simulink model "planta_PROTEC_fornalha_LC"  (Simulink 8.8)
settings: Solver=ode3  StartTime=0.0  StopTime=800  FixedStep=tempo_amostragem  MaxStep=1e1  MinStep=1e-2  EnableMultiTasking=on
InitFcn:
  | planta_PROTEC_inicializacao
values from neighbouring files (symbols this model uses):
  Estado_Estacionario = [2 38.1987406965 21.9709981215 1.00092553605 3.07737941356 1.5 0.843438999559 0.0384242731301 0.118136727311 1.3 0.304251987406 0.577644341688 ... (188 elements, 1x188)]    [planta_PROTEC_estado_estacionario_inicial.mat]
  tempo_amostragem = 1e-2    (= 0.01)    [planta_PROTEC_inicializacao.m]
libraries: simulink_extras x6
(part 2 of 3)

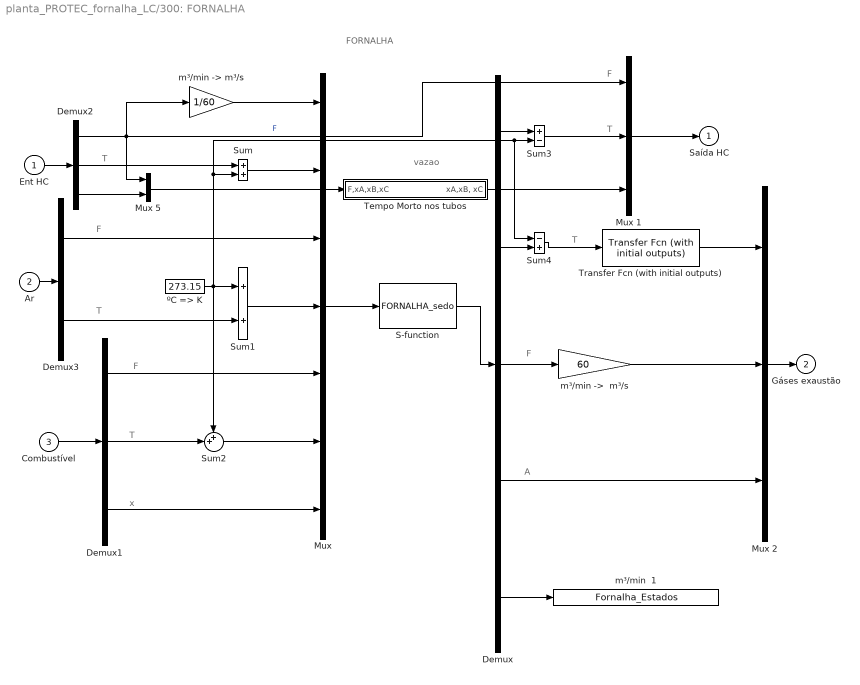
== system planta_PROTEC_fornalha_LC/300: FORNALHA ==
  note: T
  note: vazao
  note: FORNALHA
  note: T
  note: F
  note: T
  note: F
  note: A
  note: F
  note: T
  note: x
  note: F
  note: T
  Ent HC : Inport
  Ar : Inport  Port=2
  Combustível : Inport  Port=3
  "   m³/min  1" : ToWorkspace  VariableName=Fornalha_Estados  SampleTime=-1
      settings: Decimation=10
  Demux : Demux  Outputs=[ 1 1 1 1 26 ]
  Demux1 : Demux  Outputs=3
  Demux2 : Demux  Outputs=[ 1 1 3]
  Demux3 : Demux  Outputs=2
  Mux : Mux  Inputs=7
  Mux 1 : Mux  Inputs=3
  Mux 2 : Mux  Inputs=3
  Mux 5 : Mux  Inputs=[1 3]
  S-function : S-Function  FunctionName=FORNALHA_sedo  Parameters=Estado_Estacionario  SFunctionDeploymentMode=off  EnableBusSupport=off
  Sum : Sum  SaturateOnIntegerOverflow=on  InputSameDT=on  OutDataTypeStr=Inherit: Same as first input
  Sum1 : Sum  SaturateOnIntegerOverflow=on  InputSameDT=on  OutDataTypeStr=Inherit: Same as first input
  Sum2 : Sum  Inputs=++|  SaturateOnIntegerOverflow=on  InputSameDT=on  OutDataTypeStr=Inherit: Same as first input
  Sum3 : Sum  Inputs=+-  SaturateOnIntegerOverflow=on  InputSameDT=on  OutDataTypeStr=Inherit: Same as first input
  Sum4 : Sum  Inputs=-+  SaturateOnIntegerOverflow=on  InputSameDT=on  OutDataTypeStr=Inherit: Same as first input
  Tempo Morto nos tubos : Subsystem
  Transfer Fcn (with initial outputs) : simulink_extras/Additional Linear/Transfer Fcn (with initial outputs)  N=[1]  D="[1  1]"  Y0=Estado_Estacionario(40)  U0=Estado_Estacionario(40)
  "m³/min ->  m³/s" : Gain  Gain=60  SaturateOnIntegerOverflow=on  OutDataTypeStr=Inherit: Same as input  ParamDataTypeStr=Inherit: Same as input
  "m³/min -> m³/s" : Gain  Gain=1/60  SaturateOnIntegerOverflow=on  OutDataTypeStr=Inherit: Same as input  ParamDataTypeStr=Inherit: Same as input
  ºC => K : Constant  Value=273.15
  Saída HC : Outport
  Gáses exaustão : Outport  Port=2
  wires:
  S-function/1 -> Demux/1
  Mux/1 -> S-function/1
  ºC => K/1 -> Sum1/1, Sum2/1, Sum/2, Sum3/2, Sum4/1
  Sum2/1 -> Mux/6
  Sum1/1 -> Mux/4
  Sum/1 -> Mux/2
  Demux3/2 -> Sum1/2
  Demux1/2 -> Sum2/2
  Demux1/3 -> Mux/7
  Demux/1 -> Sum3/1
  Demux/2 -> Sum4/2
  Sum3/1 -> Mux 1/2
  Mux 1/1 -> Saída HC/1
  Sum4/1 -> Transfer Fcn (with initial outputs)/1
  Mux 2/1 -> Gáses exaustão/1
  Demux/4 -> Mux 2/3
  Demux/3 -> "m³/min ->  m³/s"/1
  Demux3/1 -> Mux/3
  Demux1/1 -> Mux/5
  Ent HC/1 -> Demux2/1
  Demux2/1 -> Mux 5/1, "m³/min -> m³/s"/1, Mux 1/1  "F"
  Tempo Morto nos tubos/1("xA,xB, xC") -> Mux 1/3
  Demux2/3 -> Mux 5/2
  Mux 5/1 -> Tempo Morto nos tubos/1(F,xA,xB,xC)
  Demux2/2 -> Sum/1
  Demux/5 -> "   m³/min  1"/1
  Transfer Fcn (with initial outputs)/1 -> Mux 2/1
  "m³/min -> m³/s"/1 -> Mux/1
  "m³/min ->  m³/s"/1 -> Mux 2/2
  Combustível/1 -> Demux1/1
  Ar/1 -> Demux3/1

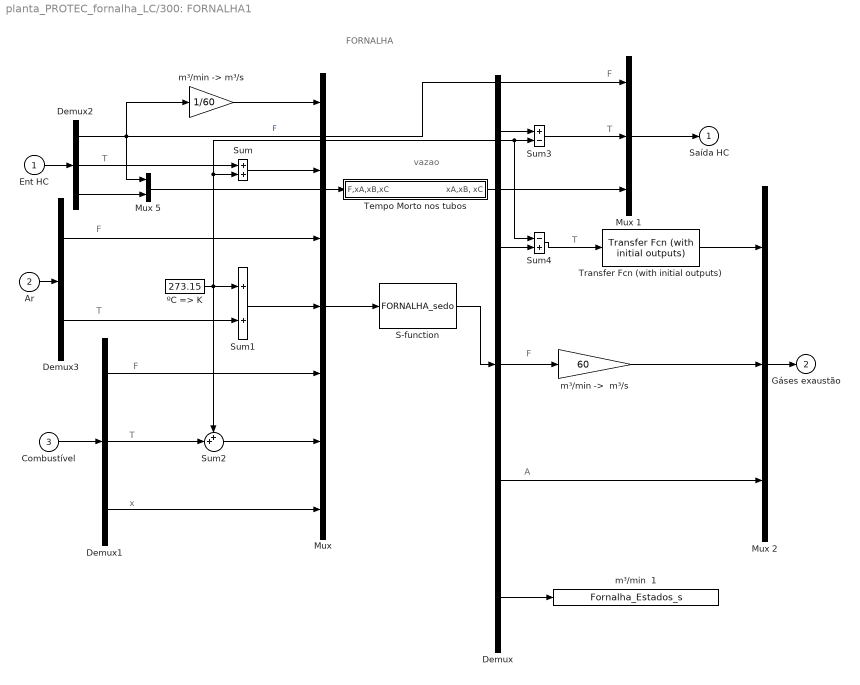
== system planta_PROTEC_fornalha_LC/300: FORNALHA1 ==
  note: T
  note: F
  note: x
  note: T
  note: F
  note: A
  note: F
  note: T
  note: F
  note: T
  note: FORNALHA
  note: vazao
  note: T
  Ent HC : Inport
  Ar : Inport  Port=2
  Combustível : Inport  Port=3
  "   m³/min  1" : ToWorkspace  VariableName=Fornalha_Estados_s  SampleTime=-1
      settings: Decimation=10
  Demux : Demux  Outputs=[ 1 1 1 1 26 ]
  Demux1 : Demux  Outputs=3
  Demux2 : Demux  Outputs=[ 1 1 3]
  Demux3 : Demux  Outputs=2
  Mux : Mux  Inputs=7
  Mux 1 : Mux  Inputs=3
  Mux 2 : Mux  Inputs=3
  Mux 5 : Mux  Inputs=[1 3]
  S-function : S-Function  FunctionName=FORNALHA_sedo  Parameters=Estado_Estacionario  SFunctionDeploymentMode=off  EnableBusSupport=off
  Sum : Sum  SaturateOnIntegerOverflow=on  InputSameDT=on  OutDataTypeStr=Inherit: Same as first input
  Sum1 : Sum  SaturateOnIntegerOverflow=on  InputSameDT=on  OutDataTypeStr=Inherit: Same as first input
  Sum2 : Sum  Inputs=++|  SaturateOnIntegerOverflow=on  InputSameDT=on  OutDataTypeStr=Inherit: Same as first input
  Sum3 : Sum  Inputs=+-  SaturateOnIntegerOverflow=on  InputSameDT=on  OutDataTypeStr=Inherit: Same as first input
  Sum4 : Sum  Inputs=-+  SaturateOnIntegerOverflow=on  InputSameDT=on  OutDataTypeStr=Inherit: Same as first input
  Tempo Morto nos tubos : Subsystem
  Transfer Fcn (with initial outputs) : simulink_extras/Additional Linear/Transfer Fcn (with initial outputs)  N=[1]  D="[1  1]"  Y0=Estado_Estacionario(40)  U0=Estado_Estacionario(40)
  "m³/min ->  m³/s" : Gain  Gain=60  SaturateOnIntegerOverflow=on  OutDataTypeStr=Inherit: Same as input  ParamDataTypeStr=Inherit: Same as input
  "m³/min -> m³/s" : Gain  Gain=1/60  SaturateOnIntegerOverflow=on  OutDataTypeStr=Inherit: Same as input  ParamDataTypeStr=Inherit: Same as input
  ºC => K : Constant  Value=273.15
  Saída HC : Outport
  Gáses exaustão : Outport  Port=2
  wires:
  Ar/1 -> Demux3/1
  Combustível/1 -> Demux1/1
  "m³/min ->  m³/s"/1 -> Mux 2/2
  "m³/min -> m³/s"/1 -> Mux/1
  Transfer Fcn (with initial outputs)/1 -> Mux 2/1
  Demux/5 -> "   m³/min  1"/1
  Demux2/2 -> Sum/1
  Mux 5/1 -> Tempo Morto nos tubos/1(F,xA,xB,xC)
  Demux2/3 -> Mux 5/2
  Tempo Morto nos tubos/1("xA,xB, xC") -> Mux 1/3
  Demux2/1 -> Mux 1/1, "m³/min -> m³/s"/1, Mux 5/1  "F"
  Ent HC/1 -> Demux2/1
  Demux1/1 -> Mux/5
  Demux3/1 -> Mux/3
  Demux/3 -> "m³/min ->  m³/s"/1
  Demux/4 -> Mux 2/3
  Mux 2/1 -> Gáses exaustão/1
  Sum4/1 -> Transfer Fcn (with initial outputs)/1
  Mux 1/1 -> Saída HC/1
  Sum3/1 -> Mux 1/2
  Demux/2 -> Sum4/2
  Demux/1 -> Sum3/1
  Demux1/3 -> Mux/7
  Demux1/2 -> Sum2/2
  Demux3/2 -> Sum1/2
  Sum/1 -> Mux/2
  Sum1/1 -> Mux/4
  Sum2/1 -> Mux/6
  ºC => K/1 -> Sum4/1, Sum3/2, Sum/2, Sum2/1, Sum1/1
  Mux/1 -> S-function/1
  S-function/1 -> Demux/1

== system planta_PROTEC_fornalha_LC/B 1 ==
  note: Bomba
  Sinal de entrada : Inport
  Sinal de saída : Outport
  wires:
  Sinal de entrada/1 -> Sinal de saída/1

== system planta_PROTEC_fornalha_LC/B 303 ==
  note: Bomba
  Sinal de entrada : Inport
  Sinal de saída : Outport
  wires:
  Sinal de entrada/1 -> Sinal de saída/1

== system planta_PROTEC_fornalha_LC/Clique duas vezes sobre  "?" para obter maiores informações  ==
  note: Autores:
      | Noaldo Leite Silva
      | Rômulo
  note: TROCADOR BITUBULAR EM CONTRA-CORRENTE.
      | Para rodar primeiro clique duas vezes no quadro que reinicializa os dados.
  note: Fonte:
  note: Simulação de uma fornalha
  note: Fonte: PROCESS CONTROL MODULES. Francis Doyle III
  note: Simulação de uma caldeira
  note: Fonte: Pellegrinetti, Gordon and Bentsman, Joseph. Nonlinear Control Oriented Boiler Modeling -
      | A Benchmark Problem for Controller Design. IEEE Transactions on Control System Technology,
      | Vol. 4, No. 1, January 1996
  note: Modelo do CSTR adaptado do Corripio, pg 471 a 474.
  note: Sugestões e críticas enviar para
      | e-mail: kalid@ufba.br
      |
      | Departamento de Engenharia Química da UFBA
      | Tel: (71) 3203.9811   ou   (71) 9188.3316
      |
      | Arquivos e outras informações em
      |
      | www.PEI.ufba.br
  note: Simulação de uma coluna de destilação
      | Fonte: S. Skogestad and M. Morari,
      | "Understanding the Dynamic Behavior of Distillation Columns'',
      | Ind. & Eng. Chem. Research, 27, 10, 1848-1862 (1988)
  note: Itens a desenvolver:
      | 1 Coluna de destilação: efeito da variação de pressão na separação
      | 2 Coluna de destilação: efeito da variação de pressão do vapor na entalpia do vapor para o refervedor
      | 3 Coluna de destilação: modelo fenomenológico com 3 componentes
      | 4 Ventilador de ar para fornalha
      | 5 Controle de pH no tanque de efluente
      | 6 Sistema de tratamento biológico no efluente
      | 7 No destilado instalar reator tubular
      | 8 Compressor de H2 e CO para reator tubular
      | 9 Melhor modelo de transferêcia de calor dos gases de exaustão na caldeira e no reator CSTR
      | 10 Modelo fenomenológico de bombas, ventiladores e exaustores
      | 11 Modelo fenomenológico de compressores

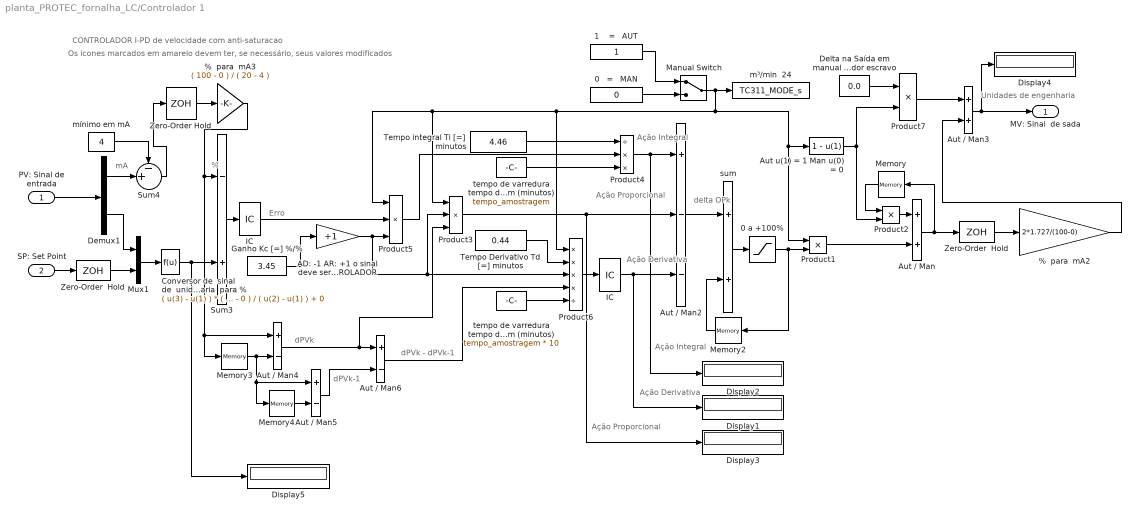
== system planta_PROTEC_fornalha_LC/Controlador 1 ==
  note: Ação
      | Proporcional
  note: Ação
      | Derivativa
  note: Ação
      | Integral
  note: Unidades
      | de
      | engenharia
  note: Ação
      | Integral
  note: Ação
      | Derivativa
  note: dPVk - dPVk-1
  note: dPVk
  note: dPVk-1
  note: delta
      | OPk
  note: Ação
      | Proporcional
  note: %
  note: mA
  note: CONTROLADOR I-PD de velocidade com anti-saturacao
  note: Os ícones marcados em amarelo devem ter, se necessário, seus valores modificados
  note: Erro
  PV: Sinal de entrada : Inport
  SP: Set Point : Inport  Port=2
  "   m³/min  24" : ToWorkspace  VariableName=TC311_MODE_s  SampleTime=-1
      settings: Decimation=10
  "  1    =   AUT" : Constant
  " IC" : InitialCondition  Value=0
  %  para  mA2 : Gain  Gain=2*1.727/(100-0)  SaturateOnIntegerOverflow=on  OutDataTypeStr=Inherit: Same as input  ParamDataTypeStr=Inherit: Same as input
  %  para  mA3 : Gain  Gain=( 100 - 0 ) / ( 20 - 4 )  SaturateOnIntegerOverflow=on  OutDataTypeStr=Inherit: Same as input  ParamDataTypeStr=Inherit: Same as input
  0   =   MAN : Constant  Value=0
  0 a +100% : Saturate  UpperLimit=100  LowerLimit=0  LinearizeAsGain=off
  "AD: -1 AR: +1 o sinal deve ser modificado para a  correta  AÇÃO  DO  CONTROLADOR   " : Gain  Gain=+1  SaturateOnIntegerOverflow=on  OutDataTypeStr=Inherit: Same as input  ParamDataTypeStr=Inherit: Same as input
  Aut / Man : Sum  SaturateOnIntegerOverflow=on  InputSameDT=on  OutDataTypeStr=Inherit: Same as first input
  Aut / Man2 : Sum  Inputs=+--  SaturateOnIntegerOverflow=on  InputSameDT=on  OutDataTypeStr=Inherit: Same as first input
  Aut / Man3 : Sum  SaturateOnIntegerOverflow=on  InputSameDT=on  OutDataTypeStr=Inherit: Same as first input
  Aut / Man4 : Sum  Inputs=+-  SaturateOnIntegerOverflow=on  InputSameDT=on  OutDataTypeStr=Inherit: Same as first input
  Aut / Man5 : Sum  Inputs=+-  SaturateOnIntegerOverflow=on  InputSameDT=on  OutDataTypeStr=Inherit: Same as first input
  Aut / Man6 : Sum  Inputs=+-  SaturateOnIntegerOverflow=on  InputSameDT=on  OutDataTypeStr=Inherit: Same as first input
  Aut u(1) = 1 Man u(0) = 0 : Fcn  Expr=1 - u(1)
  Conversor de  sinal de  unidades  de  engenharia  para % : Fcn  Expr=( u(3) - u(1) ) * ( 100 - 0 ) / ( u(2) - u(1) ) + 0
  Delta na Saída em manual do controlador [=] unidades de engenharia do SP do controlador escravo : Constant  Value=0.0
  Demux1 : Demux  Outputs=[ 1 2 ]
  Display{1..5} (5 alike) : Display
  Ganho Kc [=] %/% : Constant  Value=3.45
  IC : InitialCondition  Value=0
  Manual Switch : ManualSwitch
  Memory{,2..4} (4 alike) : Memory  X0=50  InheritSampleTime=on
  Mux1 : Mux  Inputs=[ 2 1 ]
  Product1 : Product  SaturateOnIntegerOverflow=on  RndMeth=Zero  InputSameDT=on  OutDataTypeStr=Inherit: Same as first input
  Product2 : Product  SaturateOnIntegerOverflow=on  RndMeth=Zero  InputSameDT=on  OutDataTypeStr=Inherit: Same as first input
  Product3 : Product  Inputs=3  SaturateOnIntegerOverflow=on  RndMeth=Zero  InputSameDT=on  OutDataTypeStr=Inherit: Same as first input
  Product4 : Product  Inputs=/**  SaturateOnIntegerOverflow=on  RndMeth=Zero  InputSameDT=on  OutDataTypeStr=Inherit: Same as first input
  Product5 : Product  Inputs=3  SaturateOnIntegerOverflow=on  RndMeth=Zero  InputSameDT=on  OutDataTypeStr=Inherit: Same as first input
  Product6 : Product  Inputs=****/  SaturateOnIntegerOverflow=on  RndMeth=Zero  InputSameDT=on  OutDataTypeStr=Inherit: Same as first input
  Product7 : Product  SaturateOnIntegerOverflow=on  RndMeth=Zero  InputSameDT=on  OutDataTypeStr=Inherit: Same as first input
  Sum3 : Sum  Inputs=-+  SaturateOnIntegerOverflow=on  InputSameDT=on  OutDataTypeStr=Inherit: Same as first input
  Sum4 : Sum  Inputs=-+|  SaturateOnIntegerOverflow=on  InputSameDT=on  OutDataTypeStr=Inherit: Same as first input
  Tempo Derivativo Td [=] minutos : Constant  Value=0.44
  Tempo integral Ti [=] minutos : Constant  Value=4.46
  Zero-Order  Hold : ZeroOrderHold  SampleTime=tempo_amostragem
  "Zero-Order  Hold " : ZeroOrderHold  SampleTime=tempo_amostragem
  "Zero-Order Hold " : ZeroOrderHold  SampleTime=tempo_amostragem
  mínimo em mA : Constant  Value=4
  sum : Sum  SaturateOnIntegerOverflow=on  InputSameDT=on  OutDataTypeStr=Inherit: Same as first input
  tempo de varredura tempo de amostragem (minutos) : Constant  Value=tempo_amostragem
  "tempo de varredura tempo de amostragem (minutos) " : Constant  Value=tempo_amostragem * 10
  MV: Sinal  de sada : Outport
  wires:
  Tempo Derivativo Td [=] minutos/1 -> Product6/2
  0   =   MAN/1 -> Manual Switch/2
  "  1    =   AUT"/1 -> Manual Switch/1
  Zero-Order  Hold/1 -> Mux1/2
  Demux1/2 -> Mux1/1
  Mux1/1 -> Conversor de  sinal de  unidades  de  engenharia  para %/1
  Aut / Man3/1 -> Display4/1, MV: Sinal  de sada/1
  %  para  mA2/1 -> Aut / Man3/2
  Product7/1 -> Aut / Man3/1
  Delta na Saída em manual do controlador [=] unidades de engenharia do SP do controlador escravo/1 -> Product7/1
  "Zero-Order  Hold "/1 -> %  para  mA2/1
  Sum4/1 -> "Zero-Order Hold "/1
  "Zero-Order Hold "/1 -> %  para  mA3/1
  Product3/1 -> Display3/1, Aut / Man2/2
  "AD: -1 AR: +1 o sinal deve ser modificado para a  correta  AÇÃO  DO  CONTROLADOR   "/1 -> Product5/3, Product3/2, Product6/3
  " IC"/1 -> Display1/1, Aut / Man2/3
  "tempo de varredura tempo de amostragem (minutos) "/1 -> Product6/5
  Aut / Man5/1 -> Aut / Man6/2
  Aut / Man4/1 -> Product3/3, Aut / Man6/1
  Conversor de  sinal de  unidades  de  engenharia  para %/1 -> Display5/1, Sum3/2
  Product6/1 -> " IC"/1
  Aut / Man6/1 -> Product6/4
  Memory4/1 -> Aut / Man5/2
  Memory3/1 -> Aut / Man4/2, Aut / Man5/1, Memory4/1
  Ganho Kc [=] %/%/1 -> "AD: -1 AR: +1 o sinal deve ser modificado para a  correta  AÇÃO  DO  CONTROLADOR   "/1
  IC/1 -> Product5/2
  0 a +100%/1 -> Product1/2, Memory2/1
  Memory2/1 -> sum/2
  sum/1 -> 0 a +100%/1
  Aut / Man2/1 -> sum/1
  Product4/1 -> Display2/1, Aut / Man2/1
  tempo de varredura tempo de amostragem (minutos)/1 -> Product4/3
  Tempo integral Ti [=] minutos/1 -> Product4/1
  Memory/1 -> Product2/1
  Aut / Man/1 -> "Zero-Order  Hold "/1, Memory/1
  Aut u(1) = 1 Man u(0) = 0/1 -> Product7/2, Product2/2
  Product2/1 -> Aut / Man/1
  Product1/1 -> Aut / Man/2
  Manual Switch/1 -> "   m³/min  24"/1, Product3/1, Product5/1, Product6/1, Aut u(1) = 1 Man u(0) = 0/1, Product1/1
  Product5/1 -> Product4/2
  Sum3/1 -> IC/1
  mínimo em mA/1 -> Sum4/1
  Demux1/1 -> Sum4/2
  %  para  mA3/1 -> Memory3/1, Aut / Man4/1, Sum3/1
  SP: Set Point/1 -> Zero-Order  Hold/1
  PV: Sinal de entrada/1 -> Demux1/1

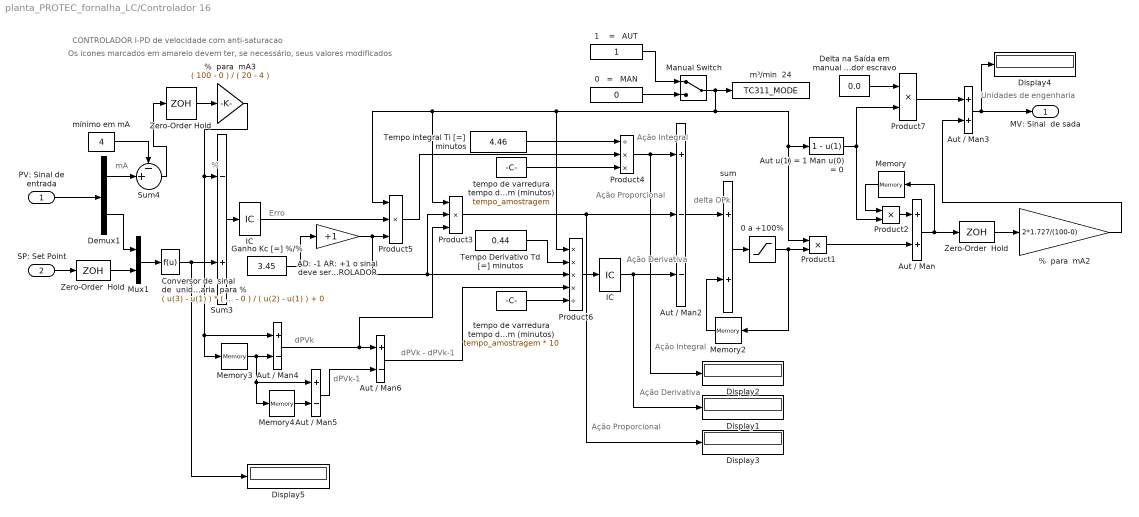
== system planta_PROTEC_fornalha_LC/Controlador 16 ==
  note: Erro
  note: Os ícones marcados em amarelo devem ter, se necessário, seus valores modificados
  note: CONTROLADOR I-PD de velocidade com anti-saturacao
  note: mA
  note: %
  note: Ação
      | Proporcional
  note: delta
      | OPk
  note: dPVk-1
  note: dPVk
  note: dPVk - dPVk-1
  note: Ação
      | Derivativa
  note: Ação
      | Integral
  note: Unidades
      | de
      | engenharia
  note: Ação
      | Integral
  note: Ação
      | Derivativa
  note: Ação
      | Proporcional
  PV: Sinal de entrada : Inport
  SP: Set Point : Inport  Port=2
  "   m³/min  24" : ToWorkspace  VariableName=TC311_MODE  SampleTime=-1
      settings: Decimation=10
  "  1    =   AUT" : Constant
  " IC" : InitialCondition  Value=0
  %  para  mA2 : Gain  Gain=2*1.727/(100-0)  SaturateOnIntegerOverflow=on  OutDataTypeStr=Inherit: Same as input  ParamDataTypeStr=Inherit: Same as input
  %  para  mA3 : Gain  Gain=( 100 - 0 ) / ( 20 - 4 )  SaturateOnIntegerOverflow=on  OutDataTypeStr=Inherit: Same as input  ParamDataTypeStr=Inherit: Same as input
  0   =   MAN : Constant  Value=0
  0 a +100% : Saturate  UpperLimit=100  LowerLimit=0  LinearizeAsGain=off
  "AD: -1 AR: +1 o sinal deve ser modificado para a  correta  AÇÃO  DO  CONTROLADOR   " : Gain  Gain=+1  SaturateOnIntegerOverflow=on  OutDataTypeStr=Inherit: Same as input  ParamDataTypeStr=Inherit: Same as input
  Aut / Man : Sum  SaturateOnIntegerOverflow=on  InputSameDT=on  OutDataTypeStr=Inherit: Same as first input
  Aut / Man2 : Sum  Inputs=+--  SaturateOnIntegerOverflow=on  InputSameDT=on  OutDataTypeStr=Inherit: Same as first input
  Aut / Man3 : Sum  SaturateOnIntegerOverflow=on  InputSameDT=on  OutDataTypeStr=Inherit: Same as first input
  Aut / Man4 : Sum  Inputs=+-  SaturateOnIntegerOverflow=on  InputSameDT=on  OutDataTypeStr=Inherit: Same as first input
  Aut / Man5 : Sum  Inputs=+-  SaturateOnIntegerOverflow=on  InputSameDT=on  OutDataTypeStr=Inherit: Same as first input
  Aut / Man6 : Sum  Inputs=+-  SaturateOnIntegerOverflow=on  InputSameDT=on  OutDataTypeStr=Inherit: Same as first input
  Aut u(1) = 1 Man u(0) = 0 : Fcn  Expr=1 - u(1)
  Conversor de  sinal de  unidades  de  engenharia  para % : Fcn  Expr=( u(3) - u(1) ) * ( 100 - 0 ) / ( u(2) - u(1) ) + 0
  Delta na Saída em manual do controlador [=] unidades de engenharia do SP do controlador escravo : Constant  Value=0.0
  Demux1 : Demux  Outputs=[ 1 2 ]
  Display{1..5} (5 alike) : Display
  Ganho Kc [=] %/% : Constant  Value=3.45
  IC : InitialCondition  Value=0
  Manual Switch : ManualSwitch
  Memory{,2..4} (4 alike) : Memory  X0=50  InheritSampleTime=on
  Mux1 : Mux  Inputs=[ 2 1 ]
  Product1 : Product  SaturateOnIntegerOverflow=on  RndMeth=Zero  InputSameDT=on  OutDataTypeStr=Inherit: Same as first input
  Product2 : Product  SaturateOnIntegerOverflow=on  RndMeth=Zero  InputSameDT=on  OutDataTypeStr=Inherit: Same as first input
  Product3 : Product  Inputs=3  SaturateOnIntegerOverflow=on  RndMeth=Zero  InputSameDT=on  OutDataTypeStr=Inherit: Same as first input
  Product4 : Product  Inputs=/**  SaturateOnIntegerOverflow=on  RndMeth=Zero  InputSameDT=on  OutDataTypeStr=Inherit: Same as first input
  Product5 : Product  Inputs=3  SaturateOnIntegerOverflow=on  RndMeth=Zero  InputSameDT=on  OutDataTypeStr=Inherit: Same as first input
  Product6 : Product  Inputs=****/  SaturateOnIntegerOverflow=on  RndMeth=Zero  InputSameDT=on  OutDataTypeStr=Inherit: Same as first input
  Product7 : Product  SaturateOnIntegerOverflow=on  RndMeth=Zero  InputSameDT=on  OutDataTypeStr=Inherit: Same as first input
  Sum3 : Sum  Inputs=-+  SaturateOnIntegerOverflow=on  InputSameDT=on  OutDataTypeStr=Inherit: Same as first input
  Sum4 : Sum  Inputs=-+|  SaturateOnIntegerOverflow=on  InputSameDT=on  OutDataTypeStr=Inherit: Same as first input
  Tempo Derivativo Td [=] minutos : Constant  Value=0.44
  Tempo integral Ti [=] minutos : Constant  Value=4.46
  Zero-Order  Hold : ZeroOrderHold  SampleTime=tempo_amostragem
  "Zero-Order  Hold " : ZeroOrderHold  SampleTime=tempo_amostragem
  "Zero-Order Hold " : ZeroOrderHold  SampleTime=tempo_amostragem
  mínimo em mA : Constant  Value=4
  sum : Sum  SaturateOnIntegerOverflow=on  InputSameDT=on  OutDataTypeStr=Inherit: Same as first input
  tempo de varredura tempo de amostragem (minutos) : Constant  Value=tempo_amostragem
  "tempo de varredura tempo de amostragem (minutos) " : Constant  Value=tempo_amostragem * 10
  MV: Sinal  de sada : Outport
  wires:
  PV: Sinal de entrada/1 -> Demux1/1
  SP: Set Point/1 -> Zero-Order  Hold/1
  %  para  mA3/1 -> Sum3/1, Aut / Man4/1, Memory3/1
  Demux1/1 -> Sum4/2
  mínimo em mA/1 -> Sum4/1
  Sum3/1 -> IC/1
  Product5/1 -> Product4/2
  Manual Switch/1 -> Product1/1, Aut u(1) = 1 Man u(0) = 0/1, Product6/1, Product5/1, Product3/1, "   m³/min  24"/1
  Product1/1 -> Aut / Man/2
  Product2/1 -> Aut / Man/1
  Aut u(1) = 1 Man u(0) = 0/1 -> Product2/2, Product7/2
  Aut / Man/1 -> Memory/1, "Zero-Order  Hold "/1
  Memory/1 -> Product2/1
  Tempo integral Ti [=] minutos/1 -> Product4/1
  tempo de varredura tempo de amostragem (minutos)/1 -> Product4/3
  Product4/1 -> Aut / Man2/1, Display2/1
  Aut / Man2/1 -> sum/1
  sum/1 -> 0 a +100%/1
  Memory2/1 -> sum/2
  0 a +100%/1 -> Memory2/1, Product1/2
  IC/1 -> Product5/2
  Ganho Kc [=] %/%/1 -> "AD: -1 AR: +1 o sinal deve ser modificado para a  correta  AÇÃO  DO  CONTROLADOR   "/1
  Memory3/1 -> Memory4/1, Aut / Man5/1, Aut / Man4/2
  Memory4/1 -> Aut / Man5/2
  Aut / Man6/1 -> Product6/4
  Product6/1 -> " IC"/1
  Conversor de  sinal de  unidades  de  engenharia  para %/1 -> Sum3/2, Display5/1
  Aut / Man4/1 -> Aut / Man6/1, Product3/3
  Aut / Man5/1 -> Aut / Man6/2
  "tempo de varredura tempo de amostragem (minutos) "/1 -> Product6/5
  " IC"/1 -> Aut / Man2/3, Display1/1
  "AD: -1 AR: +1 o sinal deve ser modificado para a  correta  AÇÃO  DO  CONTROLADOR   "/1 -> Product6/3, Product3/2, Product5/3
  Product3/1 -> Aut / Man2/2, Display3/1
  "Zero-Order Hold "/1 -> %  para  mA3/1
  Sum4/1 -> "Zero-Order Hold "/1
  "Zero-Order  Hold "/1 -> %  para  mA2/1
  Delta na Saída em manual do controlador [=] unidades de engenharia do SP do controlador escravo/1 -> Product7/1
  Product7/1 -> Aut / Man3/1
  %  para  mA2/1 -> Aut / Man3/2
  Aut / Man3/1 -> MV: Sinal  de sada/1, Display4/1
  Mux1/1 -> Conversor de  sinal de  unidades  de  engenharia  para %/1
  Demux1/2 -> Mux1/1
  Zero-Order  Hold/1 -> Mux1/2
  "  1    =   AUT"/1 -> Manual Switch/1
  0   =   MAN/1 -> Manual Switch/2
  Tempo Derivativo Td [=] minutos/1 -> Product6/2

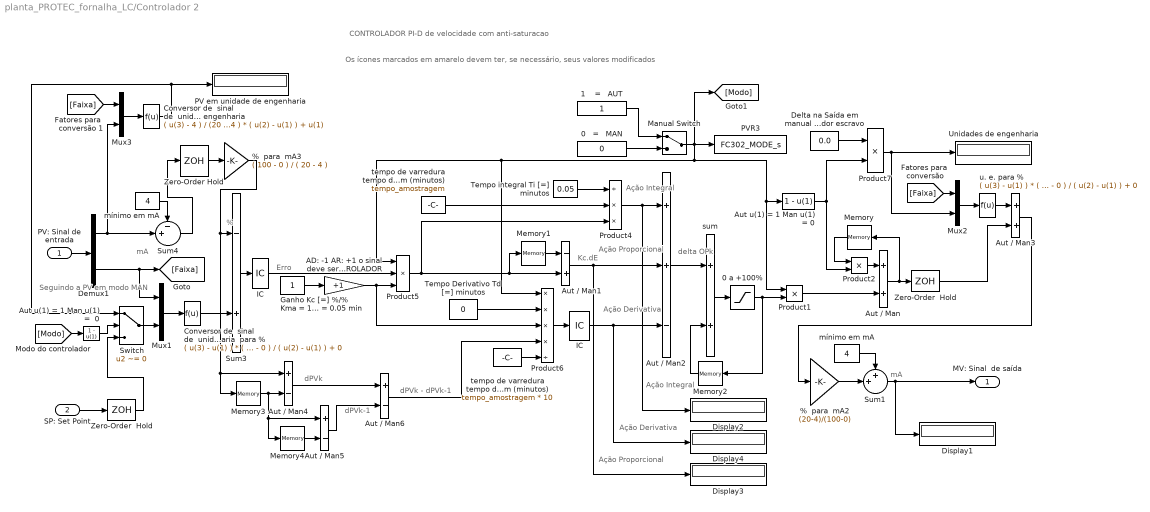
== system planta_PROTEC_fornalha_LC/Controlador 2 ==
  note: Seguindo a PV
      | em modo MAN
  note: Ação
      | Proporcional
  note: Ação
      | Derivativa
  note: Ação
      | Integral
  note: mA
  note: Erro
  note: Os ícones marcados em amarelo devem ter, se necessário, seus valores modificados
  note: CONTROLADOR PI-D de velocidade com anti-saturacao
  note: mA
  note: %
  note: Kc.dE
  note: Ação
      | Proporcional
  note: Ação
      | Integral
  note: delta
      | OPk
  note: dPVk-1
  note: dPVk
  note: dPVk - dPVk-1
  note: Ação
      | Derivativa
  PV: Sinal de entrada : Inport
  SP: Set Point : Inport  Port=2
  "  1    =   AUT" : Constant
  " IC" : InitialCondition  Value=0
  %  para  mA2 : Gain  Gain=(20-4)/(100-0)  SaturateOnIntegerOverflow=on  OutDataTypeStr=Inherit: Same as input  ParamDataTypeStr=Inherit: Same as input
  %  para  mA3 : Gain  Gain=( 100 - 0 ) / ( 20 - 4 )  SaturateOnIntegerOverflow=on  OutDataTypeStr=Inherit: Same as input  ParamDataTypeStr=Inherit: Same as input
  0   =   MAN : Constant  Value=0
  0 a +100% : Saturate  UpperLimit=100  LowerLimit=0  LinearizeAsGain=off
  "AD: -1 AR: +1 o sinal deve ser modificado para a  correta  AÇÃO  DO  CONTROLADOR  " : Gain  Gain=+1  SaturateOnIntegerOverflow=on  OutDataTypeStr=Inherit: Same as input  ParamDataTypeStr=Inherit: Same as input
  Aut / Man : Sum  SaturateOnIntegerOverflow=on  InputSameDT=on  OutDataTypeStr=Inherit: Same as first input
  Aut / Man1 : Sum  Inputs=-+  SaturateOnIntegerOverflow=on  InputSameDT=on  OutDataTypeStr=Inherit: Same as first input
  Aut / Man2 : Sum  Inputs=++-  SaturateOnIntegerOverflow=on  InputSameDT=on  OutDataTypeStr=Inherit: Same as first input
  Aut / Man3 : Sum  SaturateOnIntegerOverflow=on  InputSameDT=on  OutDataTypeStr=Inherit: Same as first input
  Aut / Man4 : Sum  Inputs=+-  SaturateOnIntegerOverflow=on  InputSameDT=on  OutDataTypeStr=Inherit: Same as first input
  Aut / Man5 : Sum  Inputs=+-  SaturateOnIntegerOverflow=on  InputSameDT=on  OutDataTypeStr=Inherit: Same as first input
  Aut / Man6 : Sum  Inputs=+-  SaturateOnIntegerOverflow=on  InputSameDT=on  OutDataTypeStr=Inherit: Same as first input
  Aut u(1) = 1 Man u(1) =  0 : Fcn  Expr=1 - u(1)
  Aut u(1) = 1 Man u(1) = 0 : Fcn  Expr=1 - u(1)
  Conversor de  sinal de  unidades  de  engenharia  para % : Fcn  Expr=( u(3) - u(1) ) * ( 100 - 0 ) / ( u(2) - u(1) ) + 0
  Conversor de  sinal de  unidades  de  mA  para  engenharia : Fcn  Expr=( u(3) - 4 ) / (20 - 4 ) * ( u(2) - u(1) ) + u(1)
  Delta na Saída em manual do controlador [=] unidades de engenharia do SP do controlador escravo : Constant  Value=0.0
  Demux1 : Demux  Outputs=[ 1 2 ]
  Display{1..4} (4 alike) : Display
  Ganho Kc [=] %/% Kma = 1 mA/mA Lambda = 0.05 min : Constant
  IC : InitialCondition  Value=0
  Manual Switch : ManualSwitch
  Memory{,2..4} (4 alike) : Memory  X0=50  InheritSampleTime=on
  Memory1 : Memory  InheritSampleTime=on
  Mux1 : Mux  Inputs=[ 2 1 ]
  Mux2 : Mux  Inputs=[ 2 1 ]
  Mux3 : Mux  Inputs=[ 2 1 ]
  PV em unidade de engenharia : Display
  PVR3 : ToWorkspace  VariableName=FC302_MODE_s  SampleTime=-1
      settings: Decimation=10
  Product1 : Product  SaturateOnIntegerOverflow=on  RndMeth=Zero  InputSameDT=on  OutDataTypeStr=Inherit: Same as first input
  Product2 : Product  SaturateOnIntegerOverflow=on  RndMeth=Zero  InputSameDT=on  OutDataTypeStr=Inherit: Same as first input
  Product4 : Product  Inputs=/**  SaturateOnIntegerOverflow=on  RndMeth=Zero  InputSameDT=on  OutDataTypeStr=Inherit: Same as first input
  Product5 : Product  Inputs=3  SaturateOnIntegerOverflow=on  RndMeth=Zero  InputSameDT=on  OutDataTypeStr=Inherit: Same as first input
  Product6 : Product  Inputs=****/  SaturateOnIntegerOverflow=on  RndMeth=Zero  InputSameDT=on  OutDataTypeStr=Inherit: Same as first input
  Product7 : Product  SaturateOnIntegerOverflow=on  RndMeth=Zero  InputSameDT=on  OutDataTypeStr=Inherit: Same as first input
  Sum1 : Sum  Inputs=++|  SaturateOnIntegerOverflow=on  InputSameDT=on  OutDataTypeStr=Inherit: Same as first input
  Sum3 : Sum  Inputs=-+  SaturateOnIntegerOverflow=on  InputSameDT=on  OutDataTypeStr=Inherit: Same as first input
  Sum4 : Sum  Inputs=-+|  SaturateOnIntegerOverflow=on  InputSameDT=on  OutDataTypeStr=Inherit: Same as first input
  Switch : Switch  Criteria=u2 ~= 0  RndMeth=Nearest  SaturateOnIntegerOverflow=on
  Tempo Derivativo Td [=] minutos : Constant  Value=0
  Tempo integral Ti [=] minutos : Constant  Value=0.05
  Unidades de engenharia : Display
  Zero-Order  Hold : ZeroOrderHold  SampleTime=tempo_amostragem
  "Zero-Order  Hold " : ZeroOrderHold  SampleTime=tempo_amostragem
  "Zero-Order Hold " : ZeroOrderHold  SampleTime=tempo_amostragem
  mínimo em mA : Constant  Value=4
  "mínimo em mA " : Constant  Value=4
  sum : Sum  SaturateOnIntegerOverflow=on  InputSameDT=on  OutDataTypeStr=Inherit: Same as first input
  tempo de varredura tempo de amostragem (minutos) : Constant  Value=tempo_amostragem
  "tempo de varredura tempo de amostragem (minutos) " : Constant  Value=tempo_amostragem * 10
  u. e. para % : Fcn  Expr=( u(3) - u(1) ) * ( 100 - 0 ) / ( u(2) - u(1) ) + 0
  MV: Sinal  de saída : Outport
  wires:
  tempo de varredura tempo de amostragem (minutos)/1 -> Product4/2
  Tempo integral Ti [=] minutos/1 -> Product4/1
  Conversor de  sinal de  unidades  de  mA  para  engenharia/1 -> PV em unidade de engenharia/1, Switch/1
  [Faixa] -> Mux3/1
  Mux3/1 -> Conversor de  sinal de  unidades  de  mA  para  engenharia/1
  Aut u(1) = 1 Man u(1) =  0/1 -> Switch/2
  Switch/1 -> Mux1/2
  [Modo] -> Aut u(1) = 1 Man u(1) =  0/1
  0   =   MAN/1 -> Manual Switch/2
  "  1    =   AUT"/1 -> Manual Switch/1
  %  para  mA2/1 -> Sum1/2
  Aut / Man3/1 -> %  para  mA2/1
  [Faixa] -> Mux2/1
  Mux2/1 -> u. e. para %/1
  Zero-Order  Hold/1 -> Aut / Man3/2
  u. e. para %/1 -> Aut / Man3/1
  "Zero-Order  Hold "/1 -> Switch/3
  Demux1/2 -> [Faixa], Mux1/1
  Product7/1 -> Mux2/2, Unidades de engenharia/1
  Delta na Saída em manual do controlador [=] unidades de engenharia do SP do controlador escravo/1 -> Product7/1
  Manual Switch/1 -> PVR3/1, [Modo], Product6/1, Product5/1, Product1/1, Aut u(1) = 1 Man u(1) = 0/1
  %  para  mA3/1 -> Sum3/1, Aut / Man4/1, Memory3/1
  "Zero-Order Hold "/1 -> %  para  mA3/1
  Sum4/1 -> "Zero-Order Hold "/1
  Sum1/1 -> Display1/1, MV: Sinal  de saída/1
  "mínimo em mA "/1 -> Sum1/1
  PV: Sinal de entrada/1 -> Demux1/1
  SP: Set Point/1 -> "Zero-Order  Hold "/1
  Mux1/1 -> Conversor de  sinal de  unidades  de  engenharia  para %/1
  Demux1/1 -> Mux3/2, Sum4/2
  mínimo em mA/1 -> Sum4/1
  Sum3/1 -> IC/1
  Product5/1 -> Product4/3, Aut / Man1/2, Memory1/1
  Product1/1 -> Aut / Man/2
  Product2/1 -> Aut / Man/1
  Aut u(1) = 1 Man u(1) = 0/1 -> Product7/2, Product2/2
  Aut / Man/1 -> Zero-Order  Hold/1, Memory/1
  Memory/1 -> Product2/1
  Memory1/1 -> Aut / Man1/1
  Product4/1 -> Display2/1, Aut / Man2/1
  Aut / Man1/1 -> Display3/1, Aut / Man2/2
  Aut / Man2/1 -> sum/1
  sum/1 -> 0 a +100%/1
  Memory2/1 -> sum/2
  0 a +100%/1 -> Memory2/1, Product1/2
  IC/1 -> Product5/2
  Ganho Kc [=] %/% Kma = 1 mA/mA Lambda = 0.05 min/1 -> "AD: -1 AR: +1 o sinal deve ser modificado para a  correta  AÇÃO  DO  CONTROLADOR  "/1
  Memory3/1 -> Memory4/1, Aut / Man5/1, Aut / Man4/2
  Memory4/1 -> Aut / Man5/2
  Aut / Man6/1 -> Product6/4
  Tempo Derivativo Td [=] minutos/1 -> Product6/2
  Product6/1 -> " IC"/1
  Conversor de  sinal de  unidades  de  engenharia  para %/1 -> Sum3/2
  Aut / Man4/1 -> Aut / Man6/1
  Aut / Man5/1 -> Aut / Man6/2
  "tempo de varredura tempo de amostragem (minutos) "/1 -> Product6/5
  " IC"/1 -> Display4/1, Aut / Man2/3
  "AD: -1 AR: +1 o sinal deve ser modificado para a  correta  AÇÃO  DO  CONTROLADOR  "/1 -> Product6/3, Product5/3

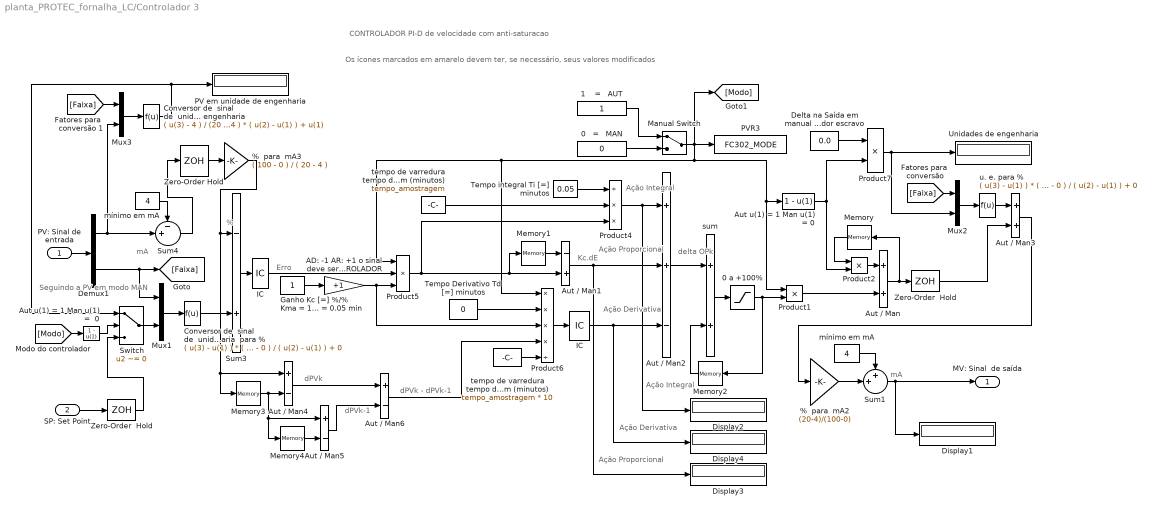
== system planta_PROTEC_fornalha_LC/Controlador 3 ==
  note: Ação
      | Derivativa
  note: dPVk - dPVk-1
  note: dPVk
  note: dPVk-1
  note: delta
      | OPk
  note: Ação
      | Integral
  note: Ação
      | Proporcional
  note: Kc.dE
  note: %
  note: mA
  note: CONTROLADOR PI-D de velocidade com anti-saturacao
  note: Os ícones marcados em amarelo devem ter, se necessário, seus valores modificados
  note: Erro
  note: mA
  note: Ação
      | Integral
  note: Ação
      | Derivativa
  note: Ação
      | Proporcional
  note: Seguindo a PV
      | em modo MAN
  PV: Sinal de entrada : Inport
  SP: Set Point : Inport  Port=2
  "  1    =   AUT" : Constant
  " IC" : InitialCondition  Value=0
  %  para  mA2 : Gain  Gain=(20-4)/(100-0)  SaturateOnIntegerOverflow=on  OutDataTypeStr=Inherit: Same as input  ParamDataTypeStr=Inherit: Same as input
  %  para  mA3 : Gain  Gain=( 100 - 0 ) / ( 20 - 4 )  SaturateOnIntegerOverflow=on  OutDataTypeStr=Inherit: Same as input  ParamDataTypeStr=Inherit: Same as input
  0   =   MAN : Constant  Value=0
  0 a +100% : Saturate  UpperLimit=100  LowerLimit=0  LinearizeAsGain=off
  "AD: -1 AR: +1 o sinal deve ser modificado para a  correta  AÇÃO  DO  CONTROLADOR  " : Gain  Gain=+1  SaturateOnIntegerOverflow=on  OutDataTypeStr=Inherit: Same as input  ParamDataTypeStr=Inherit: Same as input
  Aut / Man : Sum  SaturateOnIntegerOverflow=on  InputSameDT=on  OutDataTypeStr=Inherit: Same as first input
  Aut / Man1 : Sum  Inputs=-+  SaturateOnIntegerOverflow=on  InputSameDT=on  OutDataTypeStr=Inherit: Same as first input
  Aut / Man2 : Sum  Inputs=++-  SaturateOnIntegerOverflow=on  InputSameDT=on  OutDataTypeStr=Inherit: Same as first input
  Aut / Man3 : Sum  SaturateOnIntegerOverflow=on  InputSameDT=on  OutDataTypeStr=Inherit: Same as first input
  Aut / Man4 : Sum  Inputs=+-  SaturateOnIntegerOverflow=on  InputSameDT=on  OutDataTypeStr=Inherit: Same as first input
  Aut / Man5 : Sum  Inputs=+-  SaturateOnIntegerOverflow=on  InputSameDT=on  OutDataTypeStr=Inherit: Same as first input
  Aut / Man6 : Sum  Inputs=+-  SaturateOnIntegerOverflow=on  InputSameDT=on  OutDataTypeStr=Inherit: Same as first input
  Aut u(1) = 1 Man u(1) =  0 : Fcn  Expr=1 - u(1)
  Aut u(1) = 1 Man u(1) = 0 : Fcn  Expr=1 - u(1)
  Conversor de  sinal de  unidades  de  engenharia  para % : Fcn  Expr=( u(3) - u(1) ) * ( 100 - 0 ) / ( u(2) - u(1) ) + 0
  Conversor de  sinal de  unidades  de  mA  para  engenharia : Fcn  Expr=( u(3) - 4 ) / (20 - 4 ) * ( u(2) - u(1) ) + u(1)
  Delta na Saída em manual do controlador [=] unidades de engenharia do SP do controlador escravo : Constant  Value=0.0
  Demux1 : Demux  Outputs=[ 1 2 ]
  Display{1..4} (4 alike) : Display
  Ganho Kc [=] %/% Kma = 1 mA/mA Lambda = 0.05 min : Constant
  IC : InitialCondition  Value=0
  Manual Switch : ManualSwitch
  Memory{,2..4} (4 alike) : Memory  X0=50  InheritSampleTime=on
  Memory1 : Memory  InheritSampleTime=on
  Mux1 : Mux  Inputs=[ 2 1 ]
  Mux2 : Mux  Inputs=[ 2 1 ]
  Mux3 : Mux  Inputs=[ 2 1 ]
  PV em unidade de engenharia : Display
  PVR3 : ToWorkspace  VariableName=FC302_MODE  SampleTime=-1
      settings: Decimation=10
  Product1 : Product  SaturateOnIntegerOverflow=on  RndMeth=Zero  InputSameDT=on  OutDataTypeStr=Inherit: Same as first input
  Product2 : Product  SaturateOnIntegerOverflow=on  RndMeth=Zero  InputSameDT=on  OutDataTypeStr=Inherit: Same as first input
  Product4 : Product  Inputs=/**  SaturateOnIntegerOverflow=on  RndMeth=Zero  InputSameDT=on  OutDataTypeStr=Inherit: Same as first input
  Product5 : Product  Inputs=3  SaturateOnIntegerOverflow=on  RndMeth=Zero  InputSameDT=on  OutDataTypeStr=Inherit: Same as first input
  Product6 : Product  Inputs=****/  SaturateOnIntegerOverflow=on  RndMeth=Zero  InputSameDT=on  OutDataTypeStr=Inherit: Same as first input
  Product7 : Product  SaturateOnIntegerOverflow=on  RndMeth=Zero  InputSameDT=on  OutDataTypeStr=Inherit: Same as first input
  Sum1 : Sum  Inputs=++|  SaturateOnIntegerOverflow=on  InputSameDT=on  OutDataTypeStr=Inherit: Same as first input
  Sum3 : Sum  Inputs=-+  SaturateOnIntegerOverflow=on  InputSameDT=on  OutDataTypeStr=Inherit: Same as first input
  Sum4 : Sum  Inputs=-+|  SaturateOnIntegerOverflow=on  InputSameDT=on  OutDataTypeStr=Inherit: Same as first input
  Switch : Switch  Criteria=u2 ~= 0  RndMeth=Nearest  SaturateOnIntegerOverflow=on
  Tempo Derivativo Td [=] minutos : Constant  Value=0
  Tempo integral Ti [=] minutos : Constant  Value=0.05
  Unidades de engenharia : Display
  Zero-Order  Hold : ZeroOrderHold  SampleTime=tempo_amostragem
  "Zero-Order  Hold " : ZeroOrderHold  SampleTime=tempo_amostragem
  "Zero-Order Hold " : ZeroOrderHold  SampleTime=tempo_amostragem
  mínimo em mA : Constant  Value=4
  "mínimo em mA " : Constant  Value=4
  sum : Sum  SaturateOnIntegerOverflow=on  InputSameDT=on  OutDataTypeStr=Inherit: Same as first input
  tempo de varredura tempo de amostragem (minutos) : Constant  Value=tempo_amostragem
  "tempo de varredura tempo de amostragem (minutos) " : Constant  Value=tempo_amostragem * 10
  u. e. para % : Fcn  Expr=( u(3) - u(1) ) * ( 100 - 0 ) / ( u(2) - u(1) ) + 0
  MV: Sinal  de saída : Outport
  wires:
  "AD: -1 AR: +1 o sinal deve ser modificado para a  correta  AÇÃO  DO  CONTROLADOR  "/1 -> Product5/3, Product6/3
  " IC"/1 -> Aut / Man2/3, Display4/1
  "tempo de varredura tempo de amostragem (minutos) "/1 -> Product6/5
  Aut / Man5/1 -> Aut / Man6/2
  Aut / Man4/1 -> Aut / Man6/1
  Conversor de  sinal de  unidades  de  engenharia  para %/1 -> Sum3/2
  Product6/1 -> " IC"/1
  Tempo Derivativo Td [=] minutos/1 -> Product6/2
  Aut / Man6/1 -> Product6/4
  Memory4/1 -> Aut / Man5/2
  Memory3/1 -> Aut / Man4/2, Aut / Man5/1, Memory4/1
  Ganho Kc [=] %/% Kma = 1 mA/mA Lambda = 0.05 min/1 -> "AD: -1 AR: +1 o sinal deve ser modificado para a  correta  AÇÃO  DO  CONTROLADOR  "/1
  IC/1 -> Product5/2
  0 a +100%/1 -> Product1/2, Memory2/1
  Memory2/1 -> sum/2
  sum/1 -> 0 a +100%/1
  Aut / Man2/1 -> sum/1
  Aut / Man1/1 -> Aut / Man2/2, Display3/1
  Product4/1 -> Aut / Man2/1, Display2/1
  Memory1/1 -> Aut / Man1/1
  Memory/1 -> Product2/1
  Aut / Man/1 -> Memory/1, Zero-Order  Hold/1
  Aut u(1) = 1 Man u(1) = 0/1 -> Product2/2, Product7/2
  Product2/1 -> Aut / Man/1
  Product1/1 -> Aut / Man/2
  Product5/1 -> Memory1/1, Aut / Man1/2, Product4/3
  Sum3/1 -> IC/1
  mínimo em mA/1 -> Sum4/1
  Demux1/1 -> Sum4/2, Mux3/2
  Mux1/1 -> Conversor de  sinal de  unidades  de  engenharia  para %/1
  SP: Set Point/1 -> "Zero-Order  Hold "/1
  PV: Sinal de entrada/1 -> Demux1/1
  "mínimo em mA "/1 -> Sum1/1
  Sum1/1 -> MV: Sinal  de saída/1, Display1/1
  Sum4/1 -> "Zero-Order Hold "/1
  "Zero-Order Hold "/1 -> %  para  mA3/1
  %  para  mA3/1 -> Memory3/1, Aut / Man4/1, Sum3/1
  Manual Switch/1 -> Aut u(1) = 1 Man u(1) = 0/1, Product1/1, Product5/1, Product6/1, [Modo], PVR3/1
  Delta na Saída em manual do controlador [=] unidades de engenharia do SP do controlador escravo/1 -> Product7/1
  Product7/1 -> Unidades de engenharia/1, Mux2/2
  Demux1/2 -> Mux1/1, [Faixa]
  "Zero-Order  Hold "/1 -> Switch/3
  u. e. para %/1 -> Aut / Man3/1
  Zero-Order  Hold/1 -> Aut / Man3/2
  Mux2/1 -> u. e. para %/1
  [Faixa] -> Mux2/1
  Aut / Man3/1 -> %  para  mA2/1
  %  para  mA2/1 -> Sum1/2
  "  1    =   AUT"/1 -> Manual Switch/1
  0   =   MAN/1 -> Manual Switch/2
  [Modo] -> Aut u(1) = 1 Man u(1) =  0/1
  Switch/1 -> Mux1/2
  Aut u(1) = 1 Man u(1) =  0/1 -> Switch/2
  Mux3/1 -> Conversor de  sinal de  unidades  de  mA  para  engenharia/1
  [Faixa] -> Mux3/1
  Conversor de  sinal de  unidades  de  mA  para  engenharia/1 -> Switch/1, PV em unidade de engenharia/1
  Tempo integral Ti [=] minutos/1 -> Product4/1
  tempo de varredura tempo de amostragem (minutos)/1 -> Product4/2

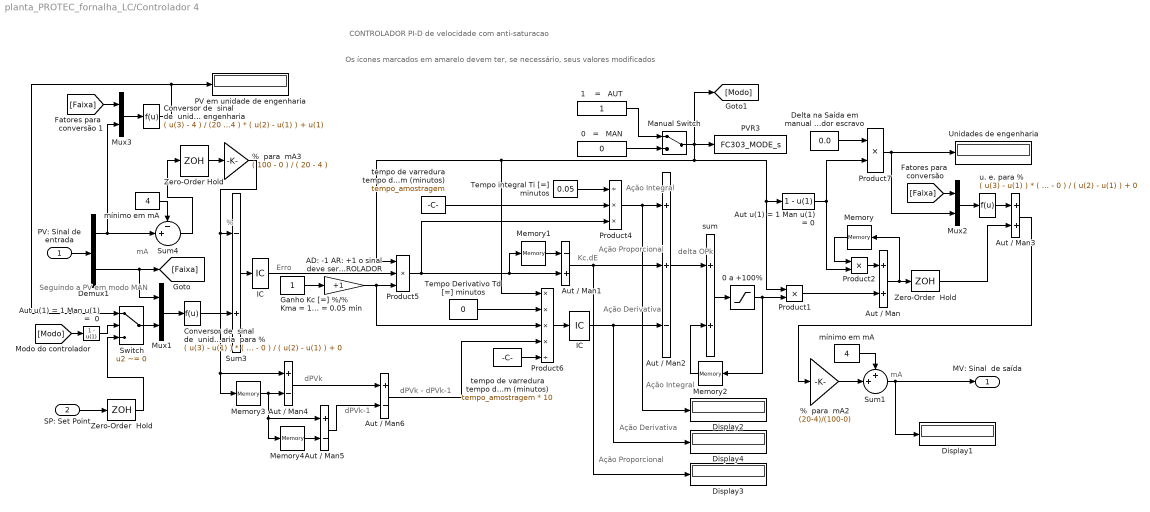
== system planta_PROTEC_fornalha_LC/Controlador 4 ==
  note: Seguindo a PV
      | em modo MAN
  note: Ação
      | Proporcional
  note: Ação
      | Derivativa
  note: Ação
      | Integral
  note: mA
  note: Erro
  note: Os ícones marcados em amarelo devem ter, se necessário, seus valores modificados
  note: CONTROLADOR PI-D de velocidade com anti-saturacao
  note: mA
  note: %
  note: Kc.dE
  note: Ação
      | Proporcional
  note: Ação
      | Integral
  note: delta
      | OPk
  note: dPVk-1
  note: dPVk
  note: dPVk - dPVk-1
  note: Ação
      | Derivativa
  PV: Sinal de entrada : Inport
  SP: Set Point : Inport  Port=2
  "  1    =   AUT" : Constant
  " IC" : InitialCondition  Value=0
  %  para  mA2 : Gain  Gain=(20-4)/(100-0)  SaturateOnIntegerOverflow=on  OutDataTypeStr=Inherit: Same as input  ParamDataTypeStr=Inherit: Same as input
  %  para  mA3 : Gain  Gain=( 100 - 0 ) / ( 20 - 4 )  SaturateOnIntegerOverflow=on  OutDataTypeStr=Inherit: Same as input  ParamDataTypeStr=Inherit: Same as input
  0   =   MAN : Constant  Value=0
  0 a +100% : Saturate  UpperLimit=100  LowerLimit=0  LinearizeAsGain=off
  "AD: -1 AR: +1 o sinal deve ser modificado para a  correta  AÇÃO  DO  CONTROLADOR  " : Gain  Gain=+1  SaturateOnIntegerOverflow=on  OutDataTypeStr=Inherit: Same as input  ParamDataTypeStr=Inherit: Same as input
  Aut / Man : Sum  SaturateOnIntegerOverflow=on  InputSameDT=on  OutDataTypeStr=Inherit: Same as first input
  Aut / Man1 : Sum  Inputs=-+  SaturateOnIntegerOverflow=on  InputSameDT=on  OutDataTypeStr=Inherit: Same as first input
  Aut / Man2 : Sum  Inputs=++-  SaturateOnIntegerOverflow=on  InputSameDT=on  OutDataTypeStr=Inherit: Same as first input
  Aut / Man3 : Sum  SaturateOnIntegerOverflow=on  InputSameDT=on  OutDataTypeStr=Inherit: Same as first input
  Aut / Man4 : Sum  Inputs=+-  SaturateOnIntegerOverflow=on  InputSameDT=on  OutDataTypeStr=Inherit: Same as first input
  Aut / Man5 : Sum  Inputs=+-  SaturateOnIntegerOverflow=on  InputSameDT=on  OutDataTypeStr=Inherit: Same as first input
  Aut / Man6 : Sum  Inputs=+-  SaturateOnIntegerOverflow=on  InputSameDT=on  OutDataTypeStr=Inherit: Same as first input
  Aut u(1) = 1 Man u(1) =  0 : Fcn  Expr=1 - u(1)
  Aut u(1) = 1 Man u(1) = 0 : Fcn  Expr=1 - u(1)
  Conversor de  sinal de  unidades  de  engenharia  para % : Fcn  Expr=( u(3) - u(1) ) * ( 100 - 0 ) / ( u(2) - u(1) ) + 0
  Conversor de  sinal de  unidades  de  mA  para  engenharia : Fcn  Expr=( u(3) - 4 ) / (20 - 4 ) * ( u(2) - u(1) ) + u(1)
  Delta na Saída em manual do controlador [=] unidades de engenharia do SP do controlador escravo : Constant  Value=0.0
  Demux1 : Demux  Outputs=[ 1 2 ]
  Display{1..4} (4 alike) : Display
  Ganho Kc [=] %/% Kma = 1 mA/mA Lambda = 0.05 min : Constant
  IC : InitialCondition  Value=0
  Manual Switch : ManualSwitch
  Memory{,2..4} (4 alike) : Memory  X0=50  InheritSampleTime=on
  Memory1 : Memory  InheritSampleTime=on
  Mux1 : Mux  Inputs=[ 2 1 ]
  Mux2 : Mux  Inputs=[ 2 1 ]
  Mux3 : Mux  Inputs=[ 2 1 ]
  PV em unidade de engenharia : Display
  PVR3 : ToWorkspace  VariableName=FC303_MODE_s  SampleTime=-1
      settings: Decimation=10
  Product1 : Product  SaturateOnIntegerOverflow=on  RndMeth=Zero  InputSameDT=on  OutDataTypeStr=Inherit: Same as first input
  Product2 : Product  SaturateOnIntegerOverflow=on  RndMeth=Zero  InputSameDT=on  OutDataTypeStr=Inherit: Same as first input
  Product4 : Product  Inputs=/**  SaturateOnIntegerOverflow=on  RndMeth=Zero  InputSameDT=on  OutDataTypeStr=Inherit: Same as first input
  Product5 : Product  Inputs=3  SaturateOnIntegerOverflow=on  RndMeth=Zero  InputSameDT=on  OutDataTypeStr=Inherit: Same as first input
  Product6 : Product  Inputs=****/  SaturateOnIntegerOverflow=on  RndMeth=Zero  InputSameDT=on  OutDataTypeStr=Inherit: Same as first input
  Product7 : Product  SaturateOnIntegerOverflow=on  RndMeth=Zero  InputSameDT=on  OutDataTypeStr=Inherit: Same as first input
  Sum1 : Sum  Inputs=++|  SaturateOnIntegerOverflow=on  InputSameDT=on  OutDataTypeStr=Inherit: Same as first input
  Sum3 : Sum  Inputs=-+  SaturateOnIntegerOverflow=on  InputSameDT=on  OutDataTypeStr=Inherit: Same as first input
  Sum4 : Sum  Inputs=-+|  SaturateOnIntegerOverflow=on  InputSameDT=on  OutDataTypeStr=Inherit: Same as first input
  Switch : Switch  Criteria=u2 ~= 0  RndMeth=Nearest  SaturateOnIntegerOverflow=on
  Tempo Derivativo Td [=] minutos : Constant  Value=0
  Tempo integral Ti [=] minutos : Constant  Value=0.05
  Unidades de engenharia : Display
  Zero-Order  Hold : ZeroOrderHold  SampleTime=tempo_amostragem
  "Zero-Order  Hold " : ZeroOrderHold  SampleTime=tempo_amostragem
  "Zero-Order Hold " : ZeroOrderHold  SampleTime=tempo_amostragem
  mínimo em mA : Constant  Value=4
  "mínimo em mA " : Constant  Value=4
  sum : Sum  SaturateOnIntegerOverflow=on  InputSameDT=on  OutDataTypeStr=Inherit: Same as first input
  tempo de varredura tempo de amostragem (minutos) : Constant  Value=tempo_amostragem
  "tempo de varredura tempo de amostragem (minutos) " : Constant  Value=tempo_amostragem * 10
  u. e. para % : Fcn  Expr=( u(3) - u(1) ) * ( 100 - 0 ) / ( u(2) - u(1) ) + 0
  MV: Sinal  de saída : Outport
  wires:
  tempo de varredura tempo de amostragem (minutos)/1 -> Product4/2
  Tempo integral Ti [=] minutos/1 -> Product4/1
  Conversor de  sinal de  unidades  de  mA  para  engenharia/1 -> PV em unidade de engenharia/1, Switch/1
  [Faixa] -> Mux3/1
  Mux3/1 -> Conversor de  sinal de  unidades  de  mA  para  engenharia/1
  Aut u(1) = 1 Man u(1) =  0/1 -> Switch/2
  Switch/1 -> Mux1/2
  [Modo] -> Aut u(1) = 1 Man u(1) =  0/1
  0   =   MAN/1 -> Manual Switch/2
  "  1    =   AUT"/1 -> Manual Switch/1
  %  para  mA2/1 -> Sum1/2
  Aut / Man3/1 -> %  para  mA2/1
  [Faixa] -> Mux2/1
  Mux2/1 -> u. e. para %/1
  Zero-Order  Hold/1 -> Aut / Man3/2
  u. e. para %/1 -> Aut / Man3/1
  "Zero-Order  Hold "/1 -> Switch/3
  Demux1/2 -> [Faixa], Mux1/1
  Product7/1 -> Mux2/2, Unidades de engenharia/1
  Delta na Saída em manual do controlador [=] unidades de engenharia do SP do controlador escravo/1 -> Product7/1
  Manual Switch/1 -> PVR3/1, [Modo], Product6/1, Product5/1, Product1/1, Aut u(1) = 1 Man u(1) = 0/1
  %  para  mA3/1 -> Sum3/1, Aut / Man4/1, Memory3/1
  "Zero-Order Hold "/1 -> %  para  mA3/1
  Sum4/1 -> "Zero-Order Hold "/1
  Sum1/1 -> Display1/1, MV: Sinal  de saída/1
  "mínimo em mA "/1 -> Sum1/1
  PV: Sinal de entrada/1 -> Demux1/1
  SP: Set Point/1 -> "Zero-Order  Hold "/1
  Mux1/1 -> Conversor de  sinal de  unidades  de  engenharia  para %/1
  Demux1/1 -> Mux3/2, Sum4/2
  mínimo em mA/1 -> Sum4/1
  Sum3/1 -> IC/1
  Product5/1 -> Product4/3, Aut / Man1/2, Memory1/1
  Product1/1 -> Aut / Man/2
  Product2/1 -> Aut / Man/1
  Aut u(1) = 1 Man u(1) = 0/1 -> Product7/2, Product2/2
  Aut / Man/1 -> Zero-Order  Hold/1, Memory/1
  Memory/1 -> Product2/1
  Memory1/1 -> Aut / Man1/1
  Product4/1 -> Display2/1, Aut / Man2/1
  Aut / Man1/1 -> Display3/1, Aut / Man2/2
  Aut / Man2/1 -> sum/1
  sum/1 -> 0 a +100%/1
  Memory2/1 -> sum/2
  0 a +100%/1 -> Memory2/1, Product1/2
  IC/1 -> Product5/2
  Ganho Kc [=] %/% Kma = 1 mA/mA Lambda = 0.05 min/1 -> "AD: -1 AR: +1 o sinal deve ser modificado para a  correta  AÇÃO  DO  CONTROLADOR  "/1
  Memory3/1 -> Memory4/1, Aut / Man5/1, Aut / Man4/2
  Memory4/1 -> Aut / Man5/2
  Aut / Man6/1 -> Product6/4
  Tempo Derivativo Td [=] minutos/1 -> Product6/2
  Product6/1 -> " IC"/1
  Conversor de  sinal de  unidades  de  engenharia  para %/1 -> Sum3/2
  Aut / Man4/1 -> Aut / Man6/1
  Aut / Man5/1 -> Aut / Man6/2
  "tempo de varredura tempo de amostragem (minutos) "/1 -> Product6/5
  " IC"/1 -> Display4/1, Aut / Man2/3
  "AD: -1 AR: +1 o sinal deve ser modificado para a  correta  AÇÃO  DO  CONTROLADOR  "/1 -> Product6/3, Product5/3
